simulink model "mavsim_trim"  (R2025b)
settings: Solver=ode45  StartTime=0.0  StopTime=10  RelTol=1e-3
undefined symbols (not defined in the file): forces_block
settings Model: Creator=parakh  LastModifiedBy=parakh

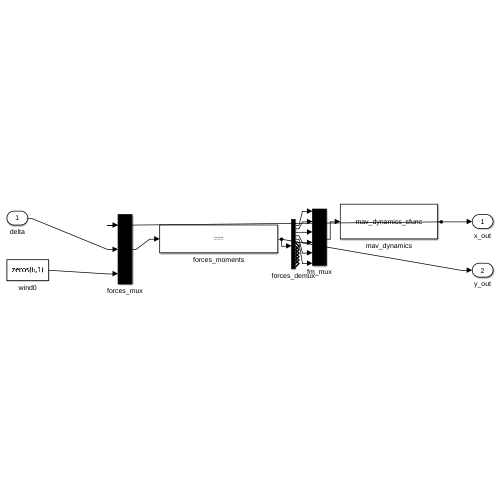
[thumbnail: Simulink's stored preview of the top-level diagram]
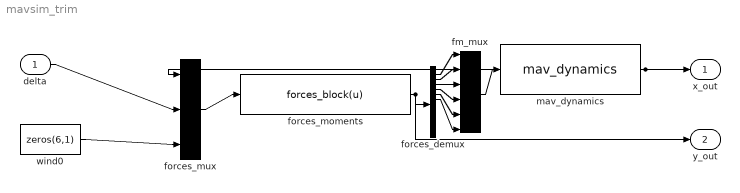
== system mavsim_trim ==
  delta : Inport  PortDimensions=4
  fm_mux : Mux  Inputs=6
  forces_demux : Demux  Outputs=12
  forces_moments : MATLABFcn  MATLABFcn=forces_block(u)  OutputDimensions=12
  forces_mux : Mux  Inputs=3
  mav_dynamics : M-S-Function  FunctionName=mav_dynamics  Parameters=P
  wind0 : Constant  Value=zeros(6,1)
  x_out : Outport
  y_out : Outport  Port=2
  wires:
  mav_dynamics/1 -> forces_mux/1, x_out/1
  delta/1 -> forces_mux/2
  wind0/1 -> forces_mux/3
  forces_mux/1 -> forces_moments/1
  forces_moments/1 -> forces_demux/1, y_out/1
  forces_demux/1 -> fm_mux/1
  forces_demux/2 -> fm_mux/2
  forces_demux/3 -> fm_mux/3
  forces_demux/4 -> fm_mux/4
  forces_demux/5 -> fm_mux/5
  forces_demux/6 -> fm_mux/6
  fm_mux/1 -> mav_dynamics/1
